simulink model "last"  (R2023b)
settings: Solver=VariableStepAuto  StartTime=0.0  StopTime=0.1  RelTol=1e-3
libraries: commdigbbndpm3 x2, dspfdesign x2, commchan3 x1, commsink2 x1, commrandsrc3 x1
settings Model: Creator=B03-402  LastModifiedBy=B03-402

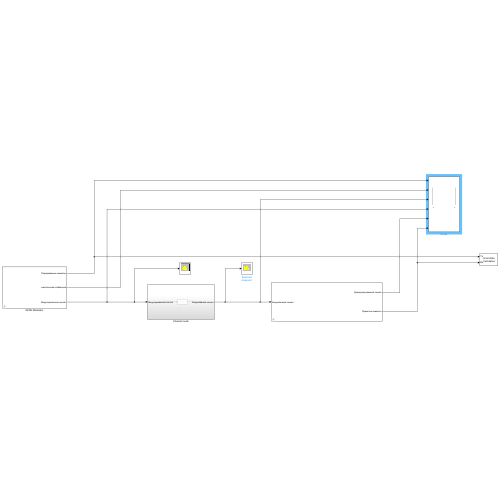
[thumbnail: Simulink's stored preview of the top-level diagram]
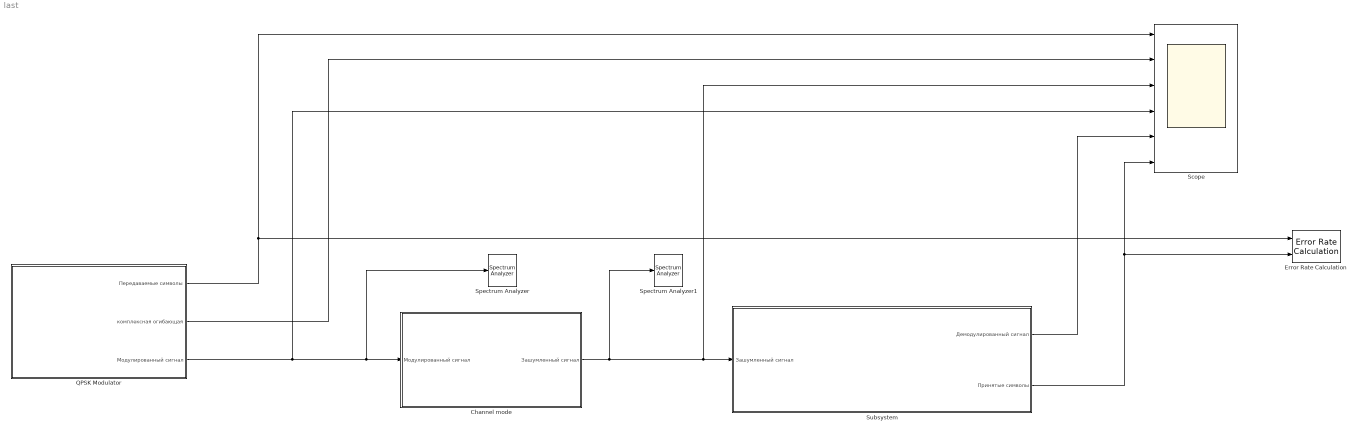
== system last ==
  Channel mode : Subsystem
  Error Rate Calculation : commsink2/Error Rate Calculation  N=2  st_delay=0  cp_mode=Entire frame  subframe=[]  PMode=Workspace  WsName=ErrorVec  RsMode2=off  stop=off  numErr=100  maxBits=1e6
      settings: LibrarySourceBlock=|
      | commhdlsink/Error Rate
      | Calculation
  QPSK Modulator : Subsystem  mask{Fc=100000, Rs=1000, fc2=10000}
      mask prompts: Fc "Частота дискртизации"; Rs "Символьная скорость"; fc2 "Частота несущей"
  Scope : Scope  NumInputPorts=6
  Spectrum Analyzer : SpectrumAnalyzer  WindowPosition=[234.000000,321.000000,800.000000,500.000000,]  Visible=on  ScopeFrameLocation=window  YLimits=[-63.56950433,18.91931285]
  Spectrum Analyzer1 : SpectrumAnalyzer  WindowPosition=[1036.000000,321.000000,800.000000,500.000000,]  Visible=on  ScopeFrameLocation=window  YLimits=[-40.63320491,16.27120725]
  Subsystem : Subsystem  mask{fc1=10000, Fc=100000, Rc=1000}
      mask prompts: fc1 "Частота несущей, Гц"; Fc "Частота дескритизаци"; Rc "Скорость символов"
  wires:
  QPSK Modulator/3(Модулированный сигнал) -> Scope/4, Spectrum Analyzer/1, Channel mode/1(Модулированный сигнал)
  Channel mode/1(Зашумленный сигнал) -> Spectrum Analyzer1/1, Scope/3, Subsystem/1(Зашумленный сигнал)
  QPSK Modulator/1(Передаваемые символы) -> Error Rate Calculation/1, Scope/1
  QPSK Modulator/2(комплексная огибающая) -> Scope/2
  Subsystem/1(Демодулированный сигнал) -> Scope/5
  Subsystem/2(Принятые символы) -> Error Rate Calculation/2, Scope/6

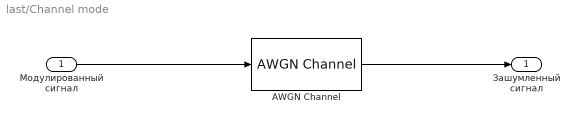
== system last/Channel mode ==
  Модулированный сигнал : Inport
  AWGN Channel : commchan3/AWGN Channel  LegacyMode=off  NoiseMethod="Signal to noise ratio  (SNR)"  noiseMode="Signal to noise ratio  (SNR)"  EbNo=10  EsNo=10  SNR=20  BitsPerSymbol=1  SignalPower=1  SamplesPerSymbol=1  SymbolPeriod=1  VarianceSource=Parameter  Variance=1  RandomStream=Global stream  Seed=67  SimulateUsing=Code generation
  Зашумленный сигнал : Outport
  wires:
  AWGN Channel/1 -> Зашумленный сигнал/1
  Модулированный сигнал/1 -> AWGN Channel/1

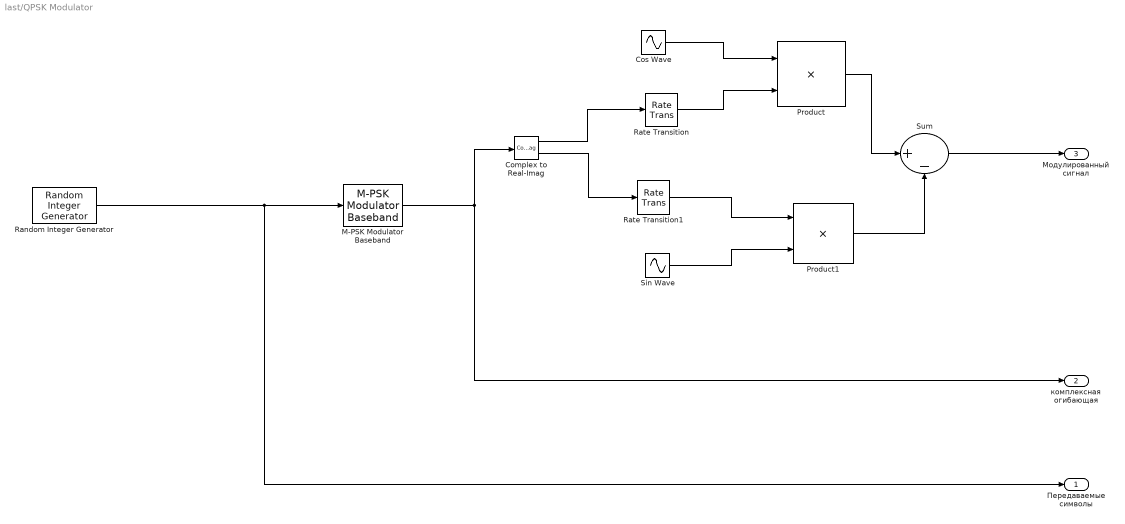
== system last/QPSK Modulator ==
  Complex to Real-Imag : ComplexToRealImag
  Cos Wave : Sin  Frequency=2*pi*fc2  Phase=pi/2  SampleTime=1/Fc
  M-PSK Modulator Baseband : commdigbbndpm3/M-PSK Modulator Baseband  M=4  InType=Integer  Enc=Gray  Mapping=[0:7]  Ph=pi/4  outDtype=double  outWordLen=16  outUDDataType=sfix(16)  outFracLenMode=Best precision  outFracLen=15  outDataTypeStr=double  outLastDataTypeStr=double
      settings: LibrarySourceBlock=|
      | commhdldigbbndpm/M-PSK
      | Modulator
      | Baseband
  Product : Product
  Product1 : Product
  Random Integer Generator : commrandsrc3/Random Integer Generator  SetSize=4  SeedSource=Auto  Seed=0  SampleTime=1/Rs  SamplesPerFrame=1  OutputDataType=double  SimulateUsing=Interpreted execution
  Rate Transition : RateTransition  OutPortSampleTime=1/Fc
  Rate Transition1 : RateTransition  OutPortSampleTime=1/Fc
  Sin Wave : Sin  Frequency=2*pi*fc2  SampleTime=1/Fc
  Sum : Sum  Inputs=|+-
  Передаваемые символы : Outport
  комплексная огибающая : Outport  Port=2
  Модулированный сигнал : Outport  Port=3
  wires:
  Complex to Real-Imag/1 -> Rate Transition/1
  Sin Wave/1 -> Product1/2
  M-PSK Modulator Baseband/1 -> комплексная огибающая/1, Complex to Real-Imag/1
  Product1/1 -> Sum/2
  Random Integer Generator/1 -> Передаваемые символы/1, M-PSK Modulator Baseband/1
  Sum/1 -> Модулированный сигнал/1
  Complex to Real-Imag/2 -> Rate Transition1/1
  Product/1 -> Sum/1
  Rate Transition/1 -> Product/2
  Cos Wave/1 -> Product/1
  Rate Transition1/1 -> Product1/1

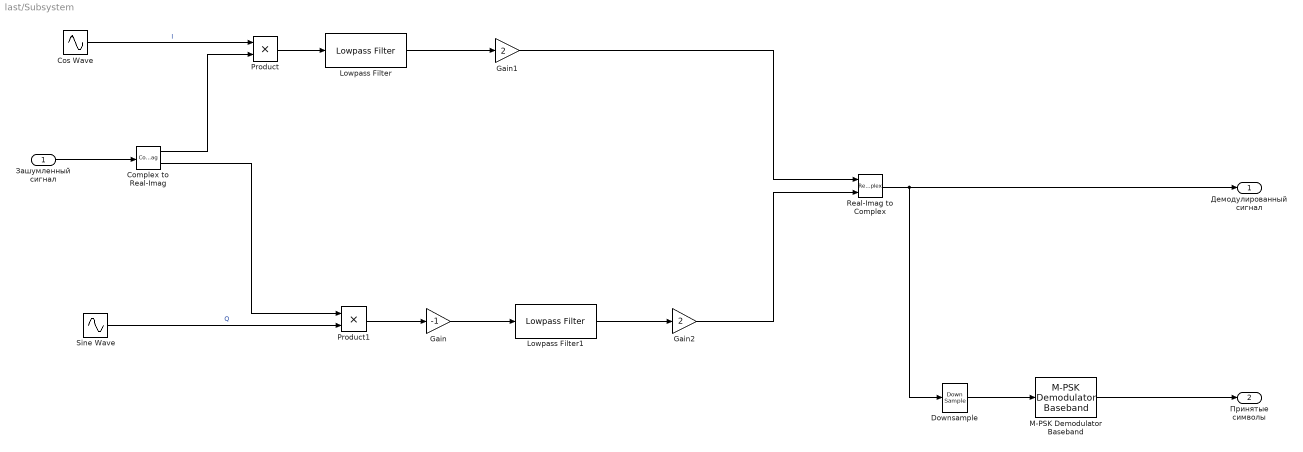
== system last/Subsystem ==
  Зашумленный сигнал : Inport
  Complex to Real-Imag : ComplexToRealImag
  Cos Wave : Sin  Frequency=2*pi*fc1  Phase=pi/2  SampleTime=1/Fc
  Downsample : DownSample  N=Fc/Rc  RateOptions=Allow multirate processing
  Gain : Gain  Gain=-1
  Gain1 : Gain  Gain=2
  Gain2 : Gain  Gain=2
  Lowpass Filter : dspfdesign/Lowpass Filter  FilterType=FIR  DesignForMinimumOrder=on  FilterOrder=50  PassbandFrequency=1000  StopbandFrequency=5000  PassbandRipple=0.1  StopbandAttenuation=80  SampleRateMode=Specify on dialog  SampleRate=Fc  SimulateUsing=Interpreted execution  roundingMode=Floor  coeffsDataTypeStr=fixdt(1,16)
  Lowpass Filter1 : dspfdesign/Lowpass Filter  FilterType=FIR  DesignForMinimumOrder=on  FilterOrder=50  PassbandFrequency=1000  StopbandFrequency=5000  PassbandRipple=0.1  StopbandAttenuation=80  SampleRateMode=Specify on dialog  SampleRate=Fc  SimulateUsing=Interpreted execution  roundingMode=Floor  coeffsDataTypeStr=fixdt(1,16)
  M-PSK Demodulator Baseband : commdigbbndpm3/M-PSK Demodulator Baseband  M=8  OutType=Integer  DecType=Hard decision  VarSource=Dialog  Variance=1  Dec=Gray  Mapping=[0:7]  Ph=pi/8  outDtype1=Inherit via internal rule  outDtype2=Inherit via internal rule  derotateFactorWordLen=16  derotateFactorDataTypeStr=Inherit: Same word length as input  derotateFactorLastDataTypeStr=Inherit: Same word length as input
  Product : Product
  Product1 : Product
  Real-Imag to Complex : RealImagToComplex
  Sine Wave : Sin  Frequency=2*pi*fc1  SampleTime=1/Fc
  Демодулированный сигнал : Outport
  Принятые символы : Outport  Port=2
  wires:
  Cos Wave/1 -> Product/1  "I"
  Sine Wave/1 -> Product1/2  "Q"
  Product/1 -> Lowpass Filter/1
  Product1/1 -> Gain/1
  Gain/1 -> Lowpass Filter1/1
  Lowpass Filter/1 -> Gain1/1
  Lowpass Filter1/1 -> Gain2/1
  Gain1/1 -> Real-Imag to Complex/1
  Gain2/1 -> Real-Imag to Complex/2
  Зашумленный сигнал/1 -> Complex to Real-Imag/1
  Complex to Real-Imag/1 -> Product/2
  Complex to Real-Imag/2 -> Product1/1
  Real-Imag to Complex/1 -> Демодулированный сигнал/1, Downsample/1
  Downsample/1 -> M-PSK Demodulator Baseband/1
  M-PSK Demodulator Baseband/1 -> Принятые символы/1
